simulink model "Continuous_System_Loop"  (R2023b)
settings: Solver=VariableStepAuto  StartTime=0.0  StopTime=10.0  RelTol=1e-3
libraries: simulink x2
settings Model: Creator=Liu  LastModifiedBy=Liu

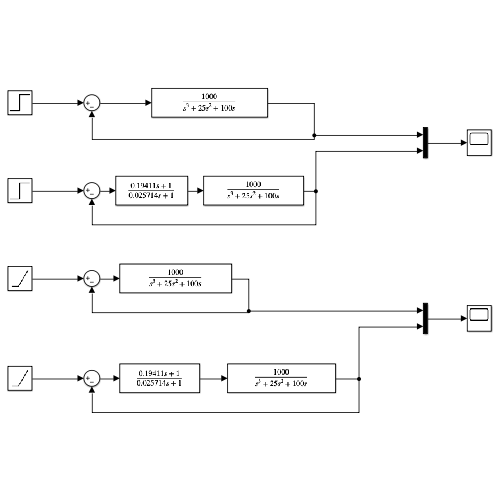
[thumbnail: Simulink's stored preview of the top-level diagram]
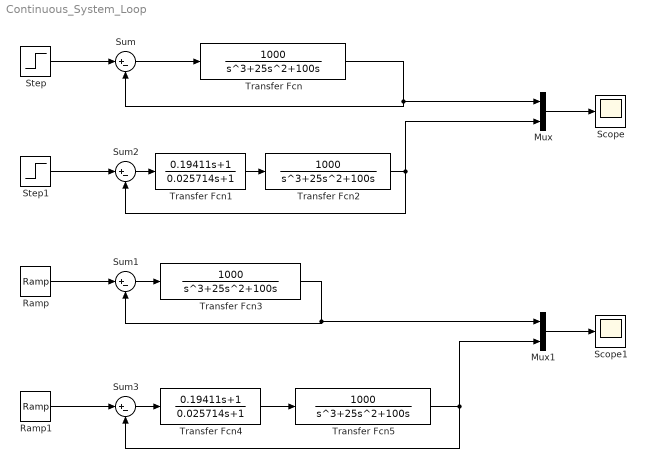
== system Continuous_System_Loop ==
  Mux : Mux  Inputs=2
  Mux1 : Mux  Inputs=2
  Ramp : simulink/Sources/Ramp  slope=1  start=0  InitialOutput=0
  Ramp1 : simulink/Sources/Ramp  slope=1  start=0  InitialOutput=0
  Scope : Scope
  Scope1 : Scope
  Step : Step  SampleTime=0
  Step1 : Step  SampleTime=0
  Sum{,1..3} (4 alike) : Sum  Inputs=|+-
  Transfer Fcn{,2..3,5} (4 alike) : TransferFcn  Numerator=[1000]  Denominator=[1 25 100 0]
  Transfer Fcn1 : TransferFcn  Numerator=[0.19411 1]  Denominator=[0.025714 1]
  Transfer Fcn4 : TransferFcn  Numerator=[0.19411 1]  Denominator=[0.025714 1]
  wires:
  Step/1 -> Sum/1
  Sum/1 -> Transfer Fcn/1
  Step1/1 -> Sum2/1
  Transfer Fcn2/1 -> Sum2/2, Mux/2
  Sum2/1 -> Transfer Fcn1/1
  Transfer Fcn1/1 -> Transfer Fcn2/1
  Mux/1 -> Scope/1
  Transfer Fcn/1 -> Sum/2, Mux/1
  Mux1/1 -> Scope1/1
  Sum1/1 -> Transfer Fcn3/1
  Transfer Fcn5/1 -> Mux1/2, Sum3/2
  Sum3/1 -> Transfer Fcn4/1
  Ramp1/1 -> Sum3/1
  Ramp/1 -> Sum1/1
  Transfer Fcn3/1 -> Mux1/1, Sum1/2
  Transfer Fcn4/1 -> Transfer Fcn5/1
